simulink model "sf_karplus_strong"  (R2025b)
settings: Solver=FixedStepDiscrete  StartTime=0.0  StopTime=10  FixedStep=0.02  RelTol=1e-3  EnableMultiTasking=on
settings Model: Creator=The MathWorks, Inc.  LastModifiedBy=The MathWorks, Inc.
settings SolverCC: AlgebraicLoopSolver=TrustRegion
settings DataIOCC: LimitDataPoints=on  ReturnWorkspaceOutputs=off
settings OptimizationCC: ReuseModelBlockBuffer=off  LifeSpan=inf
settings DebuggingCC: UnconnectedInputMsg=warning  UnconnectedOutputMsg=warning  UnconnectedLineMsg=warning  AllowSymbolicDim=off  SFUnexpectedBacktrackingDiag=warning  SFNoUnconditionalDefaultTransitionDiag=warning  SFExecutionAtInitializationDiag=none  ArithmeticOperatorsInVariantConditions=warning
settings HardwareCC: ProdBitPerPointer=32.0  ProdBitPerSizeT=32.0  ProdBitPerPtrDiffT=32.0  ProdLargestAtomicFloat=None  ProdIntDivRoundTo=Undefined  ProdEndianess=Unspecified  ProdWordSize=32.0  ProdHWDeviceType=32-bit Generic
settings ModelReferenceCC: EnableRefExpFcnMdlSchedulingChecks=on  PropagateSignalLabelsOutOfModel=off
settings SFSimCC: SimUseLocalCustomCode=off  CustomCodeUndefinedFunction=UseInterfaceOnly
settings RTWCC: RTWUseLocalCustomCode=off  GPUComputeCapability=3.5
settings CodeAppCC: StateflowObjectComments=on
settings GRTTargetCC: TargetLangStandard=C89/C90 (ANSI)
settings ConfigComp: CovMetricSettings=dw  CovSaveCumulativeToWorkspaceVar=on  CovSaveSingleToWorkspaceVar=on  CovExternalEMLEnable=off

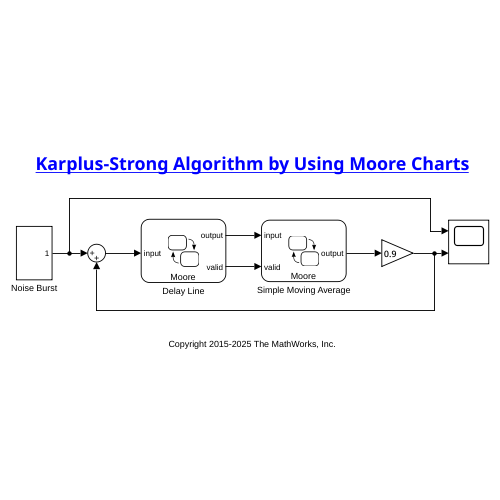
[thumbnail: Simulink's stored preview of the top-level diagram]
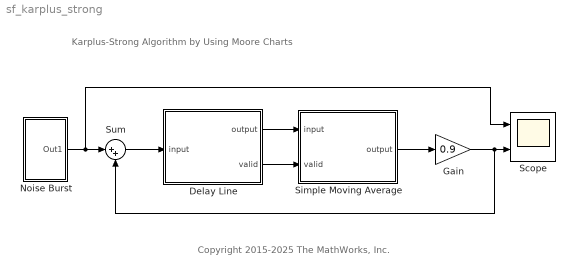
== system sf_karplus_strong ==
  note: Copyright 2015-2025 The MathWorks, Inc.
  note: Karplus-Strong Algorithm by Using Moore Charts
  Delay Line : Stateflow chart  TreatAsAtomicUnit=on
  Gain : Gain  Gain=0.9
  Noise Burst : Subsystem
  Scope : Scope  NumInputPorts=2
      settings: ActiveDisplayYMinimum=-1.23044  ActiveDisplayYMaximum=1.22791
  Simple Moving Average : Stateflow chart  TreatAsAtomicUnit=on
  Sum : Sum  Inputs=|++
  wires:
  Sum/1 -> Delay Line/1(input)
  Simple Moving Average/1(output) -> Gain/1
  Gain/1 -> Sum/2, Scope/2
  Delay Line/1(output) -> Simple Moving Average/1(input)
  Delay Line/2(" valid") -> Simple Moving Average/2(valid)
  Noise Burst/1(Out1) -> Scope/1, Sum/1

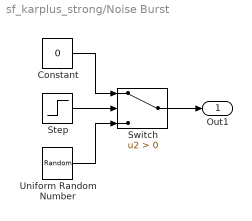
== system sf_karplus_strong/Noise Burst ==
  Constant : Constant  Value=0
  Step : Step  SampleTime=0
  Switch : Switch  Criteria=u2 > Threshold  SaturateOnIntegerOverflow=off  InputSameDT=off
  Uniform Random Number : UniformRandomNumber  SampleTime=0.02
  Out1 : Outport  VectorParamsAs1DForOutWhenUnconnected=off
  wires:
  Step/1 -> Switch/2
  Constant/1 -> Switch/1
  Uniform Random Number/1 -> Switch/3
  Switch/1 -> Out1/1

== stateflow chart sf_karplus_strong/Delay Line ==
  settings: stateMachineType=MOORE_MACHINE
  state Init
    output = 0;
    index = uint8(1);
    values = [input zeros(1,DELAY-1)];
  state y = next_index [function]
    (default) -> (junction 34) : {y = index + uint8(1);}
    (junction 34) -> (junction 35) [order 1] : [y > DELAY]
    (junction 34) -> (junction 36) [order 2]
    (junction 35) -> (junction 37) : {y = uint8(1);}
    (junction 37) -> (junction 36)
    (junction 36) -> (junction 38)
  state UnderDelayValues
    index = next_index();
    values(index) = input;
  state ShiftWindow
    output = values(next_index);
    index = next_index();
    values(index) = input;
  (default) -> Init
  Init -> UnderDelayValues
  UnderDelayValues -> ShiftWindow : after(DELAY-1, tick)
  data: y function_output; values local; input input; output output; valid output boolean; index local; DELAY constant uint8 =48

== stateflow chart sf_karplus_strong/Simple Moving Average ==
  settings: stateMachineType=MOORE_MACHINE
  state PropagateAverageToOutput [parallel]
    settings: executionOrder=1
    state SecondValid
      output = average;
    state Init
      previous = 0;
    state FirstValid
    (default) -> Init
    Init -> FirstValid : [valid]
    FirstValid -> SecondValid : [valid]
  state ComputeAverage [parallel]
    average = (input + previous)/2;
    previous = input;
    settings: executionOrder=2
  data: average local; previous local; input input; valid input; output output
